simulink model "course_lab6_lead2"  (R2024b)
settings: Solver=ode45  StartTime=0.0  StopTime=5  MaxStep=0.003333333333333334  RelTol=1e-7  AbsTol=1e-9
model workspace (MAT data in the model file):
  A = 1
  K = 10
  MpReq = 27.5
  alpha = 3
  den = [0.000154320987654 0.00814577310044 0.128565973782 1.5591167564 6.7735026919 10]
  essReq = 0.1
  frequency = 1
  num = [0 0 0 0.833333333333 5.7735026919 10]
  plant_den = [0.0166666666667 0.533333333333 1 0]
  plant_num = [0 0 0 10]
  tsReq = 1.7
  web_input = timeseries
  web_input.Name = 'unnamed'
  web_input.DataInfo = tsdata.datametadata
  web_input.DataInfo.Interpolation = tsdata.interpolation
  web_input.DataInfo.Interpolation.Fhandle : function handle (value not decoded)
  web_input.DataInfo.Interpolation.Name = 'linear'
  web_input.TimeInfo = tsdata.timemetadata
  web_input.TimeInfo.Length = 1501
  web_input.TimeInfo.DuplicateTimes = 0
  web_input.TimeInfo.Time_ = [0 0.00333333333333 0.00666666666667 0.01 0.0133333333333 0.0166666666667 0.02 0.0233333333333 0.0266666666667 0.03 0.0333333333333 0.0366666666667 ... (1501 elements, 1501x1)]
  web_input.TimeInfo.Initialized = 1
  web_input.QualityInfo = tsdata.qualmetadata
  web_input.Data_ = [1 1 1 1 1 1 1 1 1 1 1 1 ... (1501 elements, 1501x1)]
  wm = 6
  wp = 10.3923048454
  wz = 3.46410161514
settings Model: Creator=33657  LastModifiedBy=33657

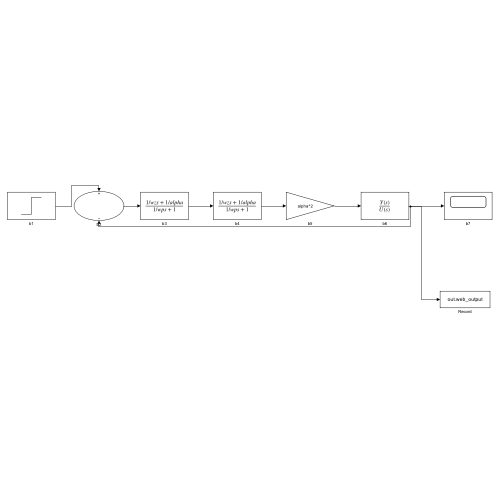
[thumbnail: Simulink's stored preview of the top-level diagram]
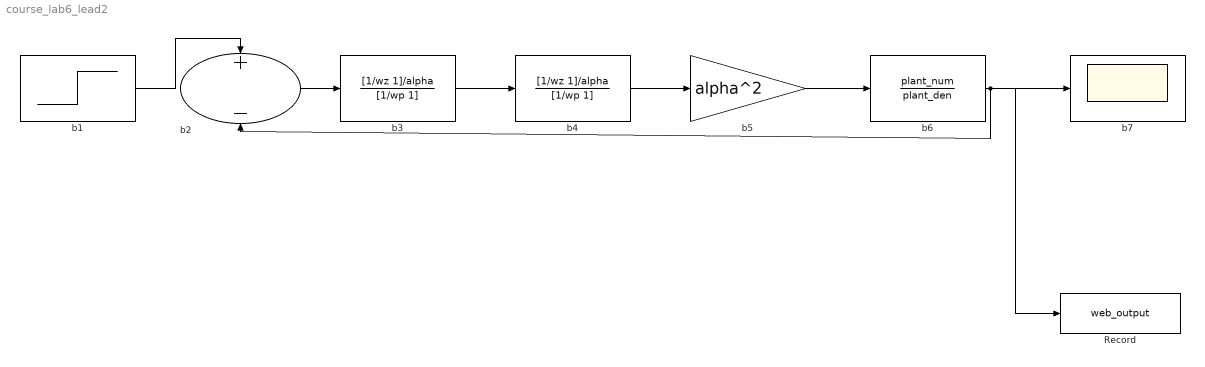
== system course_lab6_lead2 ==
  Record : ToWorkspace  VariableName=web_output  SaveFormat=Timeseries  SampleTime=-1
  b1 : Step  Time=0  After=A  SampleTime=0
  b2 : Sum  Inputs=+-
  b3 : TransferFcn  Numerator=[1/wz 1]/alpha  Denominator=[1/wp 1]
  b4 : TransferFcn  Numerator=[1/wz 1]/alpha  Denominator=[1/wp 1]
  b5 : Gain  Gain=alpha^2
  b6 : TransferFcn  Numerator=plant_num  Denominator=plant_den
  b7 : Scope
  wires:
  b1/1 -> b2/1
  b2/1 -> b3/1
  b3/1 -> b4/1
  b4/1 -> b5/1
  b5/1 -> b6/1
  b6/1 -> b2/2, b7/1, Record/1
